simulink model "sf_seqrec"  (R2025b)
settings: Solver=FixedStepDiscrete  StartTime=0.0  StopTime=10.0  RelTol=1e-3  EnableMultiTasking=on
libraries: SignalEditorBlockLib x1
Description:
  | Ref: Digital Design: From Gates to Intelligent Machines, 2006 by Bruce F. Katz
settings Model: Creator=The MathWorks, Inc.  LastModifiedBy=The MathWorks, Inc.
settings SolverCC: AlgebraicLoopSolver=TrustRegion  MaxZcPerStep=1.0
settings DataIOCC: LimitDataPoints=on  SaveFormat=Array  ReturnWorkspaceOutputs=off
settings OptimizationCC: ReuseModelBlockBuffer=off  ExpressionDepthLimit=2147483647.0  InitFltsAndDblsToZero=on  EfficientMapNaN2IntZero=off  LifeSpan=1  EfficientTunableParamExpr=on
settings DebuggingCC: SaveWithParameterizedLinksMsg=none  UnderspecifiedInitializationDetection=Classic  MergeDetectMultiDrivingBlocksExec=none  SignalResolutionControl=TryResolveAllWithWarning  SolverPrmCheckMsg=warning  FcnCallInpInsideContextMsg=warning  UnconnectedInputMsg=warning  UnconnectedOutputMsg=warning  UnconnectedLineMsg=warning  AllowSymbolicDim=off  StateNameClashWarn=warning  SFUnexpectedBacktrackingDiag=warning  SFNoUnconditionalDefaultTransitionDiag=warning  SFExecutionAtInitializationDiag=none  ArithmeticOperatorsInVariantConditions=warning
settings HardwareCC: ProdBitPerPointer=32.0  ProdBitPerSizeT=32.0  ProdBitPerPtrDiffT=32.0  ProdLargestAtomicFloat=None  ProdIntDivRoundTo=Undefined  ProdEndianess=Unspecified  ProdWordSize=32.0  ProdHWDeviceType=32-bit Generic
settings ModelReferenceCC: EnableRefExpFcnMdlSchedulingChecks=on  PropagateSignalLabelsOutOfModel=off
settings SFSimCC: SimUseLocalCustomCode=off  SimParseCustomCode=off  MATLABDynamicMemAlloc=off  CustomCodeUndefinedFunction=UseInterfaceOnly
settings RTWCC: SystemTargetFile=ert.tlc  GenCodeOnly=on  TemplateMakefile=ert_default_tmf  RTWUseLocalCustomCode=off  GPUComputeCapability=3.5  DLArmComputeVersion=19.05  Description=Real-Time Workshop Embedded Coder (no auto configuration)
settings CodeAppCC: IgnoreCustomStorageClasses=off  CustomSymbolStrGlobalVar=$N$M  CustomSymbolStrType=$N$M  CustomSymbolStrFcn=$N$M$F  CustomSymbolStrMacro=$N$M  StateflowObjectComments=on  InternalIdentifier=Classic
settings ERTTargetCC: InlinedParameterPlacement=Hierarchical  ERTCustomFileTemplate=example_file_process.tlc  ConvertIfToSwitch=off  SuppressUnreachableDefaultCases=off  TargetFcnLib=ansi_tfl_tmw.mat  MultiwordLength=2048.0  GenerateSampleERTMain=on  IncludeMdlTerminateFcn=off  SupportContinuousTime=on
settings ConfigComp: CovMetricSettings=dw  CovSaveCumulativeToWorkspaceVar=on  CovSaveSingleToWorkspaceVar=on  CovExternalEMLEnable=off  CovSFcnEnable=off

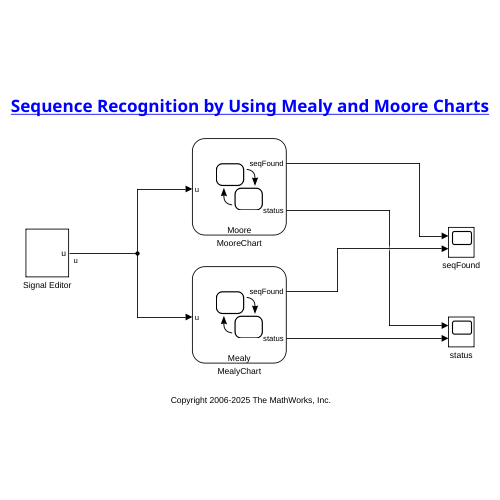
[thumbnail: Simulink's stored preview of the top-level diagram]
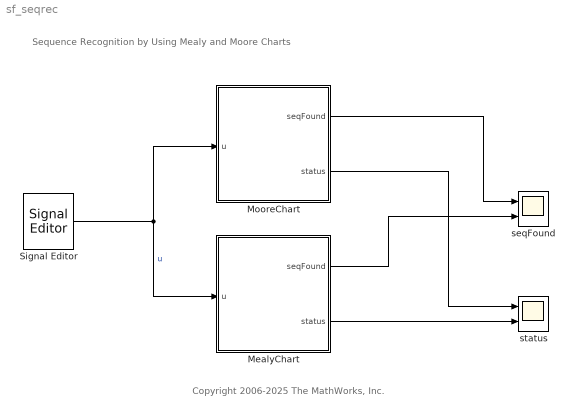
== system sf_seqrec ==
  note: Copyright 2006-2025 The MathWorks, Inc.
  note: Sequence Recognition by Using Mealy and Moore Charts
  MealyChart : Stateflow chart  TreatAsAtomicUnit=on
  MooreChart : Stateflow chart  TreatAsAtomicUnit=on
  Signal Editor : SignalEditorBlockLib/Signal Editor  FileName=SeqRecInput.mat  ActiveScenario=Group_1  ActiveSignal=u  IsBus=off  OutputBusObjectStr=Bus: BusObject  SampleTime=0  OutputAfterFinalValue=Extrapolation  Unit=inherit  PreserveSignalName=on  ApplySigPropsToAllScenarios=on  ApplySigPropsToAllSignals=off  SignalPropertySource=Dialog parameters
  seqFound : Scope  NumInputPorts=2
      settings: TimeSpan=10  Title=Moore  ActiveDisplayYMinimum=-5  ActiveDisplayYMaximum=5
  status : Scope  NumInputPorts=2
      settings: TimeSpan=10  Title=Moore  ActiveDisplayYMinimum=-5  ActiveDisplayYMaximum=5
  wires:
  Signal Editor/1 -> MealyChart/1(u), MooreChart/1(u)  "u"
  MooreChart/1(seqFound) -> seqFound/1
  MealyChart/1(seqFound) -> seqFound/2
  MealyChart/2(status) -> status/2
  MooreChart/2(status) -> status/1

== stateflow chart sf_seqrec/MooreChart ==
  settings: updateMethod=DISCRETE  sampleTime=0.5  stateMachineType=MOORE_MACHINE  executeAtInitialization=1  initializeOutput=1
  state s0
    status=0;
    seqFound=false;
  state s1
    status=1;
    seqFound=false;
  state s12
    status=2;
    seqFound=false;
  state s121
    status=3;
    seqFound=false;
  state s1213
    status=4;
    seqFound=true;
  s1213 -> s1 [order 1] : [u==1]
  s121 -> s1 [order 1] : [u==1]
  (default) -> s0
  s121 -> s12 [order 3] : [u==2]
  s1 -> s0 [order 2] : [u~=1]
  s1 -> s12 [order 1] : [u==2]
  s121 -> s1213 [order 2] : [u==3]
  s12 -> s121 [order 1] : [u==1]
  s0 -> s1 : [u==1]
  s1213 -> s0 [order 2]
  s121 -> s0 [order 4]
  s12 -> s0 [order 2]
  data: u input; seqFound output boolean; status output double

== stateflow chart sf_seqrec/MealyChart ==
  settings: updateMethod=DISCRETE  sampleTime=0.5  stateMachineType=MEALY_MACHINE  executeAtInitialization=1  initializeOutput=1
  state s0
  state s1
  state s12
  state s121
  state s1213
  s1213 -> s1 [order 1] : [u==1]...
      | {status=1;...
      | seqFound=false;}
  s121 -> s1 [order 1] : [u==1]...
      | {status=1;}
  (default) -> s0
  s121 -> s12 [order 3] : [u==2]
      | {status=2;}
  s1 -> s0 [order 2] : [u~=1]
      | {status=0;}
  s121 -> s1213 [order 2] : [u==3]
      | {status=4;
      | seqFound=true;}
  s1 -> s12 [order 1] : [u==2]
      | {status=2;}
  s12 -> s121 [order 1] : [u==1]
      | {status=3;}
  s0 -> s1 : [u==1]
      | {status=1;}
  s1213 -> s0 [order 2] : {status=0;...
      | seqFound=false;}
  s121 -> s0 [order 4] : {status=0;}
  s12 -> s0 [order 2] : {status=0;}
  data: u input; seqFound output boolean; status output double
